simulink model "y3"  (R2025b)
settings: Solver=ode15s  StartTime=0.0  StopTime=160  FixedStep=0.0001  MaxStep=0.01  RelTol=1e-6  AbsTol=1e-8
values from neighbouring files (symbols this model uses):
  A = [0  1; 1  1]    [adaptive_gamma_1000.mat]    (also in adaptive_gamma_10000.mat; adaptive_gamma_2000.mat; adaptive_nominal.mat; nonadaptive_nominal.mat)
  g_constant = 0    [adaptive_gamma_1000.mat]    (also in adaptive_gamma_10000.mat; adaptive_gamma_2000.mat; adaptive_nominal.mat)
  gamma = 1000    [adaptive_gamma_1000.mat]    (also in adaptive_gamma_10000.mat = 10000; adaptive_gamma_2000.mat = 2000; adaptive_nominal.mat)
undefined symbols (not defined in the file or in its folder): A_M, b, b_M, kappa, p12, p22, sgn
settings Model: Creator=Nickolay  LastModifiedBy=Nickolay

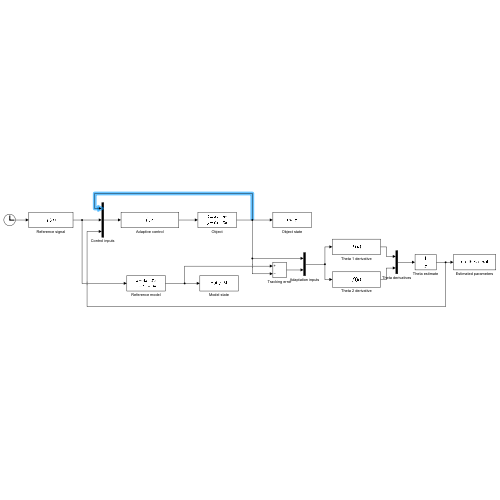
[thumbnail: Simulink's stored preview of the top-level diagram]
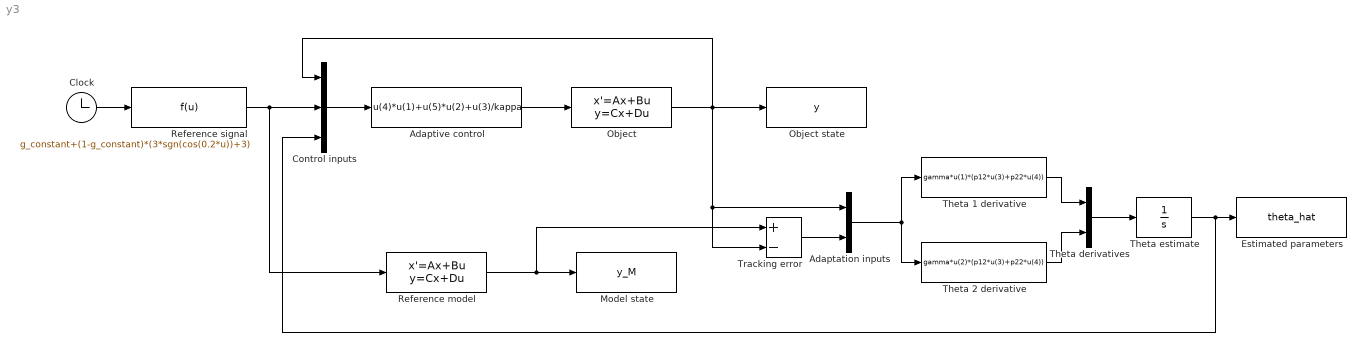
== system y3 ==
  Adaptation inputs : Mux  Inputs=2
  Adaptive control : Fcn  Expr=u(4)*u(1)+u(5)*u(2)+u(3)/kappa
  Clock : Clock
  Control inputs : Mux  Inputs=3
  Estimated parameters : ToWorkspace  VariableName=theta_hat  SaveFormat=Timeseries  SampleTime=-1
  Model state : ToWorkspace  VariableName=y_M  SaveFormat=Timeseries  SampleTime=-1
  Object : StateSpace  A=A  B=b  C=eye(2)  D=zeros(2,1)  InitialCondition=[0;0]
  Object state : ToWorkspace  VariableName=y  SaveFormat=Timeseries  SampleTime=-1
  Reference model : StateSpace  A=A_M  B=b_M  C=eye(2)  D=zeros(2,1)  InitialCondition=[0;0]
  Reference signal : Fcn  Expr=g_constant+(1-g_constant)*(3*sgn(cos(0.2*u))+3)
  Theta 1 derivative : Fcn  Expr=gamma*u(1)*(p12*u(3)+p22*u(4))
  Theta 2 derivative : Fcn  Expr=gamma*u(2)*(p12*u(3)+p22*u(4))
  Theta derivatives : Mux  Inputs=2
  Theta estimate : Integrator  InitialCondition=[0;0]
  Tracking error : Sum  Inputs=+-
  wires:
  Clock/1 -> Reference signal/1
  Control inputs/1 -> Adaptive control/1
  Adaptive control/1 -> Object/1
  Theta derivatives/1 -> Theta estimate/1
  Theta 1 derivative/1 -> Theta derivatives/1
  Theta 2 derivative/1 -> Theta derivatives/2
  Adaptation inputs/1 -> Theta 1 derivative/1, Theta 2 derivative/1
  Object/1 -> Object state/1, Tracking error/2, Adaptation inputs/1, Control inputs/1
  Reference model/1 -> Model state/1, Tracking error/1
  Tracking error/1 -> Adaptation inputs/2
  Theta estimate/1 -> Control inputs/3, Estimated parameters/1
  Reference signal/1 -> Control inputs/2, Reference model/1
